simulink model "AvonGasTurbineDgTwin"  (R2024b)
settings: Solver=VariableStepAuto  StartTime=0  StopTime=7200  FixedStep=1  RelTol=1e-3  EnableMultiTasking=on
InitFcn:
  | warning off
undefined symbols (not defined in the file or in its folder): ENV_ambient_moisture_pct, ENV_comp_inlet_press_kPa, ENV_comp_inlet_temp_C, ENV_FG_pressure_kPa, ENV_FG_temp_C
libraries: slpidlib x3, simulink x2
(part 3 of 3)

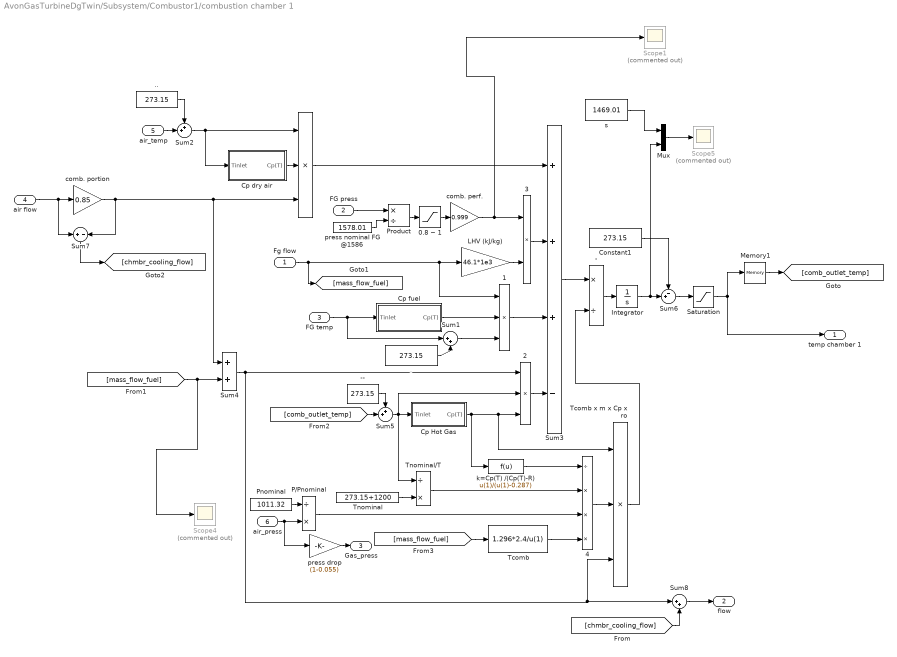
== system AvonGasTurbineDgTwin/Subsystem/Combustor1/combustion chamber 1 ==
  Fg flow : Inport
  FG press : Inport  Port=2
  FG temp : Inport  Port=3
  air flow : Inport  Port=4
  air_temp : Inport  Port=5
  air_press : Inport  Port=6
  "     " : Product  Inputs=3  RndMeth=Zero
  "     1" : Product  Inputs=3  RndMeth=Zero
  "     2" : Product  Inputs=3  RndMeth=Zero
  "     3" : Product  RndMeth=Zero
  "     4" : Product  Inputs=/***  RndMeth=Zero
  " Cp dry air " : Subsystem
  - : Product  Inputs=*/  RndMeth=Zero
  -- : Constant  Value=273.15
  . : Constant  Value=273.15
  .. : Constant  Value=273.15
  0.8 ~ 1 : Saturate  UpperLimit=1  LowerLimit=0.8
  Constant1 : Constant  Value=273.15
  "Cp Hot Gas " : Subsystem
  Cp fuel : Subsystem
  Integrator : Integrator  InitialCondition=780+273.15  LimitOutput=on  UpperSaturationLimit=2000  LowerSaturationLimit=780+273.15
  "LHV (kJ/kg) " : Gain  Gain=46.1*1e3
  Memory1 : Memory  InitialCondition=780
  Mux : Mux  Inputs=2
  P/Pnominal : Product  Inputs=/*  RndMeth=Zero
  Pnominal : Constant  Value=1011.32
  Product : Product  Inputs=*/
  Saturation : Saturate  UpperLimit=1400  LowerLimit=350
  Scope1 : Scope  Commented=on
  Scope4 : Scope  Commented=on
  Scope5 : Scope  Commented=on
  Sum1 : Sum  Inputs=|++
  Sum2 : Sum  Inputs=++|
  Sum3 : Sum  Inputs=+++-
  Sum4 : Sum  Inputs=2
  Sum5 : Sum  Inputs=++|
  Sum6 : Sum  Inputs=-+|
  Sum7 : Sum  Inputs=+-
  Sum8 : Sum  Inputs=|++
  Tcomb : Fcn  Expr=1.296*2.4/u(1)  SampleTime=1
  Tcomb x m x Cp x ro : Product  Inputs=3  RndMeth=Zero
  Tnominal : Constant  Value=273.15+1200
  Tnominal/T : Product  Inputs=/*  RndMeth=Zero
  comb. perf. : Gain  Gain=0.999
  comb. portion : Gain  Gain=0.85
  k=Cp(T) /(Cp(T)-R) : Fcn  Expr=u(1)/(u(1)-0.287)
  press drop : Gain  Gain=(1-0.055)  SampleTime=1
  press nominal FG @1586 : Constant  Value=1578.01
  s : Constant  Value=1469.01
  temp chamber 1 : Outport
  flow : Outport  Port=2
  Gas_press : Outport  Port=3
  wires:
  " Cp dry air "/1(Cp(T)) -> "     "/2
  ../1 -> Sum2/1
  Sum2/1 -> " Cp dry air "/1(Tinlet), "     "/1
  FG press/1 -> Product/1
  FG temp/1 -> Sum1/1, Cp fuel/1(Tinlet)
  Sum3/1 -> -/1
  Fg flow/1 -> "     1"/1, "LHV (kJ/kg) "/1, [mass_flow_fuel]
  Sum1/1 -> "     1"/3
  Cp fuel/1(Cp(T)) -> "     1"/2
  "     "/1 -> Sum3/1
  Memory1/1 -> [comb_outlet_temp]
  "     1"/1 -> Sum3/3
  ./1 -> Sum1/2
  "     2"/1 -> Sum3/4
  Tnominal/1 -> Tnominal/T/2
  Sum5/1 -> "     2"/2, "Cp Hot Gas "/1(Tinlet), Tnominal/T/1
  Constant1/1 -> Sum6/1
  Integrator/1 -> Mux/2, Sum6/2
  Sum6/1 -> Saturation/1
  "LHV (kJ/kg) "/1 -> "     3"/2
  Tcomb x m x Cp x ro/1 -> -/2
  Tnominal/T/1 -> "     4"/2
  [mass_flow_fuel] -> Scope4/1, Sum4/2
  "Cp Hot Gas "/1(Cp(T)) -> k=Cp(T) /(Cp(T)-R)/1, "     2"/3, Tcomb x m x Cp x ro/1
  --/1 -> Sum5/1
  Pnominal/1 -> P/Pnominal/1
  air_press/1 -> press drop/1, P/Pnominal/2
  "     4"/1 -> Tcomb x m x Cp x ro/2
  k=Cp(T) /(Cp(T)-R)/1 -> "     4"/1
  [comb_outlet_temp] -> Sum5/2
  P/Pnominal/1 -> "     4"/3
  air_temp/1 -> Sum2/2
  -/1 -> Integrator/1
  Saturation/1 -> temp chamber 1/1, Memory1/1
  s/1 -> Mux/1
  Sum4/1 -> "     2"/1, Sum8/1, Tcomb x m x Cp x ro/3
  Mux/1 -> Scope5/1
  press drop/1 -> Gas_press/1
  press nominal FG @1586/1 -> Product/2
  Product/1 -> 0.8 ~ 1/1
  0.8 ~ 1/1 -> comb. perf./1
  comb. perf./1 -> "     3"/1, Scope1/1
  "     3"/1 -> Sum3/2
  [mass_flow_fuel] -> Tcomb/1
  Tcomb/1 -> "     4"/4
  air flow/1 -> Sum7/1, comb. portion/1
  comb. portion/1 -> Sum7/2, "     "/3, Sum4/1
  Sum8/1 -> flow/1
  [chmbr_cooling_flow] -> Sum8/2
  Sum7/1 -> [chmbr_cooling_flow]

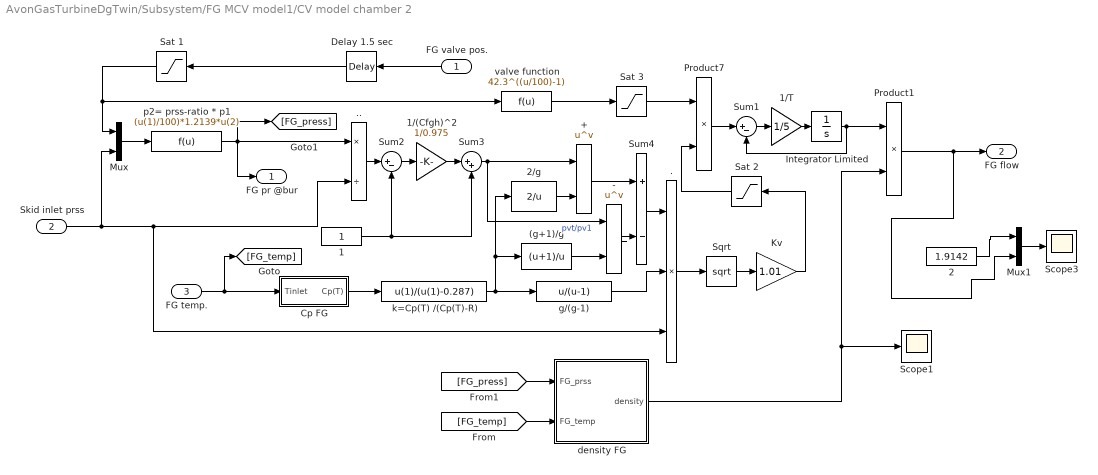
== system AvonGasTurbineDgTwin/Subsystem/FG MCV model1/CV model chamber 2 ==
  FG valve pos. : Inport
  Skid inlet prss : Inport  Port=2
  FG temp. : Inport  Port=3
  "  (g+1)/g" : Fcn  Expr=(u+1)/u
  "  Sqrt  " : Sqrt
  " k=Cp(T) /(Cp(T)-R) " : Fcn  Expr=u(1)/(u(1)-0.287)
  + : Math  Operator=pow  SignedPower=on
  - : Math  Operator=pow  SignedPower=on
  . : Product  Inputs=3  RndMeth=Zero
  .. : Product  Inputs=*/  RndMeth=Zero
  1 : Constant
  1/(Cfgh)^2 : Gain  Gain=1/0.975
  1/T : Gain  Gain=1/5
  2 : Constant  Value=1.9142
  2/g : Fcn  Expr=2/u
  Cp FG : Subsystem
  Delay 1.5 sec : TransportDelay  DelayTime=1.5  InitialOutput=30
  Integrator Limited : Integrator  InitialCondition=1.9  LimitOutput=on  UpperSaturationLimit=5  LowerSaturationLimit=0.01
  Kv : Gain  Gain=1.01
  Mux : Mux  Inputs=2
  Mux1 : Mux  Inputs=2
  Product1 : Product  RndMeth=Zero
  Product7 : Product  RndMeth=Zero
  Sat 1 : Saturate  UpperLimit=100  LowerLimit=0.01
  Sat 2 : Saturate  UpperLimit=300  LowerLimit=0.001
  Sat 3 : Saturate  UpperLimit=1  LowerLimit=0.01
  Scope1 : Scope
  Scope3 : Scope
  Sum1 : Sum  Inputs=|+-
  Sum2 : Sum  Inputs=|+-
  Sum3 : Sum  Inputs=|++
  Sum4 : Sum  Inputs=+-
  density FG : Subsystem
  g/(g-1) : Fcn  Expr=u/(u-1)
  p2= prss-ratio * p1 : Fcn  Expr=(u(1)/100)*1.2139*u(2)  SampleTime=1
  valve function : Fcn  Expr=42.3^((u/100)-1)  SampleTime=1
  FG pr @bur : Outport
  FG flow : Outport  Port=2
  wires:
  Sat 2/1 -> Product7/2
  Sum3/1 -> +/1, -/1  "pvt/pv1"
  Sum4/1 -> ./1
  "  Sqrt  "/1 -> Kv/1
  ../1 -> Sum2/1
  Skid inlet prss/1 -> ../2, ./3, Mux/2
  2/g/1 -> +/2
  1/(Cfgh)^2/1 -> Sum3/1
  Sum2/1 -> 1/(Cfgh)^2/1
  FG temp./1 -> [FG_temp], Cp FG/1(Tinlet)
  "  (g+1)/g"/1 -> -/2
  -/1 -> Sum4/2
  " k=Cp(T) /(Cp(T)-R) "/1 -> g/(g-1)/1, "  (g+1)/g"/1, 2/g/1
  g/(g-1)/1 -> ./2
  p2= prss-ratio * p1/1 -> [FG_press], ../1, FG pr @bur/1
  +/1 -> Sum4/1
  1/1 -> Sum3/2, Sum2/2
  Cp FG/1(Cp(T)) -> " k=Cp(T) /(Cp(T)-R) "/1
  Mux/1 -> p2= prss-ratio * p1/1
  valve function/1 -> Sat 3/1
  FG valve pos./1 -> Delay 1.5 sec/1
  Delay 1.5 sec/1 -> Sat 1/1
  Sat 1/1 -> Mux/1, valve function/1
  Sat 3/1 -> Product7/1
  Kv/1 -> Sat 2/1
  Sum1/1 -> 1/T/1
  1/T/1 -> Integrator Limited/1
  Integrator Limited/1 -> Product1/1, Sum1/2
  ./1 -> "  Sqrt  "/1
  Product7/1 -> Sum1/1
  [FG_temp] -> density FG/2(FG_temp)
  [FG_press] -> density FG/1(FG_prss)
  density FG/1(density) -> Scope1/1, Product1/2
  Mux1/1 -> Scope3/1
  Product1/1 -> Mux1/2, FG flow/1
  2/1 -> Mux1/1

== system AvonGasTurbineDgTwin/Subsystem/FG MCV model1/FAULT_07_FuelPrssRegulatorStuck ==
  main FG line prss : Inport
  FAULT_07_multiplier : FromWorkspace  VariableName=FAULT_07_multiplier  SampleTime=-1
  Mux : Mux  Inputs=2
  Product : Product
  Scope{,1..3} (4 alike) : Scope  Commented=on
  Out1 : Outport
  wires:
  FAULT_07_multiplier/1 -> Product/1, Scope/1
  main FG line prss/1 -> Scope1/1, Mux/2, Product/2
  Product/1 -> Mux/1, Scope2/1, Out1/1
  Mux/1 -> Scope3/1

== system AvonGasTurbineDgTwin/Subsystem/FG MCV model1/FAULT_08_FuelValveLeakage ==
  In1 : Inport
  FAULT_08_multiplier : FromWorkspace  VariableName=FAULT_08_multiplier  SampleTime=-1
  Mux : Mux  Inputs=2
  Product : Product
  Scope{,1..3} (4 alike) : Scope  Commented=on
  Out1 : Outport
  wires:
  FAULT_08_multiplier/1 -> Product/1, Scope/1
  In1/1 -> Scope1/1, Mux/2, Product/2
  Product/1 -> Mux/1, Scope2/1, Out1/1
  Mux/1 -> Scope3/1

== system AvonGasTurbineDgTwin/Subsystem/FG MCV model1/FAULT_09_FuelContamination ==
  In1 : Inport
  FAULT_09_multiplier : FromWorkspace  VariableName=FAULT_09_multiplier  SampleTime=-1
  Mux : Mux  Inputs=2
  Product : Product
  Scope{,1..3} (4 alike) : Scope  Commented=on
  Out1 : Outport
  wires:
  FAULT_09_multiplier/1 -> Product/1, Scope/1
  In1/1 -> Scope1/1, Mux/2, Product/2
  Product/1 -> Mux/1, Scope2/1, Out1/1
  Mux/1 -> Scope3/1

== system AvonGasTurbineDgTwin/Subsystem/FG MCV model1/FAULT_10_FuelLineBlockage ==
  In1 : Inport
  FAULT_10_multiplier : FromWorkspace  VariableName=FAULT_10_multiplier  SampleTime=-1
  Mux : Mux  Inputs=2
  Product : Product
  Scope{,1..3} (4 alike) : Scope  Commented=on
  Out1 : Outport
  wires:
  FAULT_10_multiplier/1 -> Product/1, Scope/1
  In1/1 -> Scope1/1, Mux/2, Product/2
  Product/1 -> Mux/1, Scope2/1, Out1/1
  Mux/1 -> Scope3/1

== system AvonGasTurbineDgTwin/Subsystem/FG MCV model1/FAULT_11_FuelPumpDegradation ==
  In1 : Inport
  FAULT_11_multiplier : FromWorkspace  VariableName=FAULT_11_multiplier  SampleTime=-1
  Mux : Mux  Inputs=2
  Product : Product
  Scope{,1..3} (4 alike) : Scope  Commented=on
  Out1 : Outport
  wires:
  FAULT_11_multiplier/1 -> Product/1, Scope/1
  In1/1 -> Scope1/1, Mux/2, Product/2
  Product/1 -> Mux/1, Scope2/1, Out1/1
  Mux/1 -> Scope3/1

== system AvonGasTurbineDgTwin/Subsystem/FG MCV model1/FAULT_12_FuelSupplyPressDrop ==
  In1 : Inport
  FAULT_12_multiplier : FromWorkspace  VariableName=FAULT_12_multiplier  SampleTime=-1
  Mux : Mux  Inputs=2
  Product : Product
  Scope{,1..3} (4 alike) : Scope  Commented=on
  Out1 : Outport
  wires:
  FAULT_12_multiplier/1 -> Product/1, Scope/1
  In1/1 -> Scope1/1, Mux/2, Product/2
  Product/1 -> Mux/1, Scope2/1, Out1/1
  Mux/1 -> Scope3/1

== system AvonGasTurbineDgTwin/Subsystem/FG MCV model1/FAULT_13_FGSupplyPressOscillation ==
  In1 : Inport
  FAULT_13_multiplier : FromWorkspace  VariableName=FAULT_13_multiplier  SampleTime=-1
  Mux : Mux  Inputs=2
  Product : Product
  Scope{,1..3} (4 alike) : Scope  Commented=on
  Out1 : Outport
  wires:
  FAULT_13_multiplier/1 -> Product/1, Scope/1
  In1/1 -> Scope1/1, Mux/2, Product/2
  Product/1 -> Mux/1, Scope2/1, Out1/1
  Mux/1 -> Scope3/1

== system AvonGasTurbineDgTwin/Subsystem/FG MCV model1/FAULT_16_FuelValveLeak ==
  FG flow : Inport
  FAULT_16_multiplier : FromWorkspace  VariableName=FAULT_16_multiplier  SampleTime=-1
  Mux : Mux  Inputs=2
  Product : Product
  Scope{,1..3} (4 alike) : Scope  Commented=on
  Out1 : Outport
  wires:
  FAULT_16_multiplier/1 -> Product/1, Scope/1
  FG flow/1 -> Scope1/1, Mux/2, Product/2
  Product/1 -> Mux/1, Scope2/1, Out1/1
  Mux/1 -> Scope3/1

== system AvonGasTurbineDgTwin/Subsystem/FG MCV model1/Subsystem1 ==
  gas prss : Inport
  FG temp. : Inport  Port=2
  FG flow : Inport  Port=3
  " 2 " : Constant  Value=2
  . : Product  Inputs=3  RndMeth=Zero
  2 : Constant  Value=2
  Kf : Gain  Gain=16.8993
  Math Function5 : Math  Operator=pow  SignedPower=on
  Memory : Memory
  Sqrt : Sqrt
  Sqrt1 : Sqrt
  Sqrt2 : Sqrt
  Sum1 : Sum  Inputs=-+|
  Sum5 : Sum  Inputs=|++
  Sum9 : Sum  Inputs=|+-
  Z : Subsystem
  c4 : Constant  Value=273.15
  n flow exp. : Constant  Value=0.4835
  pressure drop 5 kPa : Constant  Value=5
  pw : Math  Operator=pow  SignedPower=on
  pw1 : Math  Operator=pow  SignedPower=on
  " FG skid inlet prss" : Outport
  skid temp : Outport  Port=2
  wires:
  pressure drop 5 kPa/1 -> Sum1/1
  Sum1/1 -> pw1/1
  Sqrt1/1 -> ./3
  Memory/1 -> Z/2(P)
  Sqrt/1 -> ./2
  Sum5/1 -> Z/1(T), Sqrt/1
  c4/1 -> Sum5/2
  Z/1(Z) -> Sqrt1/1
  Sqrt2/1 -> Memory/1, " FG skid inlet prss"/1
  Math Function5/1 -> ./1
  FG flow/1 -> Math Function5/1
  n flow exp./1 -> Math Function5/2
  pw/1 -> Sum9/2
  2/1 -> pw/2
  Sum9/1 -> Sqrt2/1
  pw1/1 -> Sum9/1
  Kf/1 -> pw/1
  ./1 -> Kf/1
  FG temp./1 -> Sum5/1, skid temp/1
  " 2 "/1 -> pw1/2
  gas prss/1 -> Sum1/2

== system AvonGasTurbineDgTwin/Subsystem/GasGenerator/Cp @ trb. input ==
  Tinlet : Inport
  Cp : Fcn  Expr=(3.355+5.75*1e-4*u(1)-1600*u(1)^(-2))*0.28714  SampleTime=1
  Cp(T) : Outport
  wires:
  Tinlet/1 -> Cp/1
  Cp/1 -> Cp(T)/1

== system AvonGasTurbineDgTwin/Subsystem/GasGenerator/Cp @ trb. output ==
  Tinlet : Inport
  Cp : Fcn  Expr=(3.355+5.75*1e-4*u(1)-1600*u(1)^(-2))*0.28714  SampleTime=1
  Cp(T) : Outport
  wires:
  Cp/1 -> Cp(T)/1
  Tinlet/1 -> Cp/1

== system AvonGasTurbineDgTwin/Subsystem/GasGenerator/FAULT_23_GGNozzleBlockage ==
  hot_gas_flow : Inport
  FAULT_23_multiplier : FromWorkspace  VariableName=FAULT_23_multiplier  SampleTime=-1
  Mux : Mux  Inputs=2
  Product : Product
  Scope{,1..3} (4 alike) : Scope  Commented=on
  Out1 : Outport
  wires:
  FAULT_23_multiplier/1 -> Product/1, Scope/1
  hot_gas_flow/1 -> Scope1/1, Mux/2, Product/2
  Product/1 -> Mux/1, Scope2/1, Out1/1
  Mux/1 -> Scope3/1

== system AvonGasTurbineDgTwin/Subsystem/GasGenerator/FAULT_24_GGSealDegradation ==
  rotor_cooling_air_flow : Inport
  FAULT_24_multiplier : FromWorkspace  VariableName=FAULT_24_multiplier  SampleTime=-1
  Mux : Mux  Inputs=2
  Product : Product
  Scope{,1..3} (4 alike) : Scope  Commented=on
  Out1 : Outport
  wires:
  FAULT_24_multiplier/1 -> Product/1, Scope/1
  rotor_cooling_air_flow/1 -> Scope1/1, Mux/2, Product/2
  Product/1 -> Mux/1, Scope2/1, Out1/1
  Mux/1 -> Scope3/1

== system AvonGasTurbineDgTwin/Subsystem/GasGenerator/FAULT_33_SensorEnhancement ==
  In1 : Inport
  FAULT_33_multiplier : FromWorkspace  VariableName=FAULT_33_multiplier  SampleTime=-1
  Mux : Mux  Inputs=2
  Product : Product
  Scope{,1..3} (4 alike) : Scope  Commented=on
  Out1 : Outport
  wires:
  FAULT_33_multiplier/1 -> Product/1, Scope/1
  In1/1 -> Scope1/1, Mux/2, Product/2
  Product/1 -> Mux/1, Scope2/1, Out1/1
  Mux/1 -> Scope3/1

== system AvonGasTurbineDgTwin/Subsystem/GasGenerator/FAULT_34_SensorDegradation ==
  In1 : Inport
  FAULT_34_multiplier : FromWorkspace  VariableName=FAULT_34_multiplier  SampleTime=-1
  Mux : Mux  Inputs=2
  Product : Product
  Scope{,1..3} (4 alike) : Scope  Commented=on
  Out1 : Outport
  wires:
  FAULT_34_multiplier/1 -> Product/1, Scope/1
  In1/1 -> Scope1/1, Mux/2, Product/2
  Product/1 -> Mux/1, Scope2/1, Out1/1
  Mux/1 -> Scope3/1

== system AvonGasTurbineDgTwin/Subsystem/GasGenerator/FAULT_35_SensorEnhanceStep ==
  In1 : Inport
  FAULT_35_multiplier : FromWorkspace  VariableName=FAULT_35_multiplier  SampleTime=-1
  Mux : Mux  Inputs=2
  Product : Product
  Scope{,1..3} (4 alike) : Scope  Commented=on
  Out1 : Outport
  wires:
  FAULT_35_multiplier/1 -> Product/1, Scope/1
  In1/1 -> Scope1/1, Mux/2, Product/2
  Product/1 -> Mux/1, Scope2/1, Out1/1
  Mux/1 -> Scope3/1

== system AvonGasTurbineDgTwin/Subsystem/GasGenerator/FAULT_36_SensorDegradeStep ==
  In1 : Inport
  FAULT_36_multiplier : FromWorkspace  VariableName=FAULT_36_multiplier  SampleTime=-1
  Mux : Mux  Inputs=2
  Product : Product
  Scope{,1..3} (4 alike) : Scope  Commented=on
  Out1 : Outport
  wires:
  FAULT_36_multiplier/1 -> Product/1, Scope/1
  In1/1 -> Scope1/1, Mux/2, Product/2
  Product/1 -> Mux/1, Scope2/1, Out1/1
  Mux/1 -> Scope3/1

== system AvonGasTurbineDgTwin/Subsystem/GasGenerator/FAULT_37_SensorFreez ==
  temp gas : Inport
  FAULT_37_multiplier : FromWorkspace  VariableName=FAULT_37_multiplier  SampleTime=-1
  Memory : Memory  InheritSampleTime=on
  Scope{,1..3} (4 alike) : Scope  Commented=on
  Switch : Switch  Criteria=u2 > Threshold  Threshold=0.5  SaturateOnIntegerOverflow=off  InputSameDT=off
  Out1 : Outport
  wires:
  FAULT_37_multiplier/1 -> Scope3/1, Switch/2
  temp gas/1 -> Scope2/1, Switch/1
  Memory/1 -> Scope/1, Switch/3
  Switch/1 -> Scope1/1, Out1/1, Memory/1

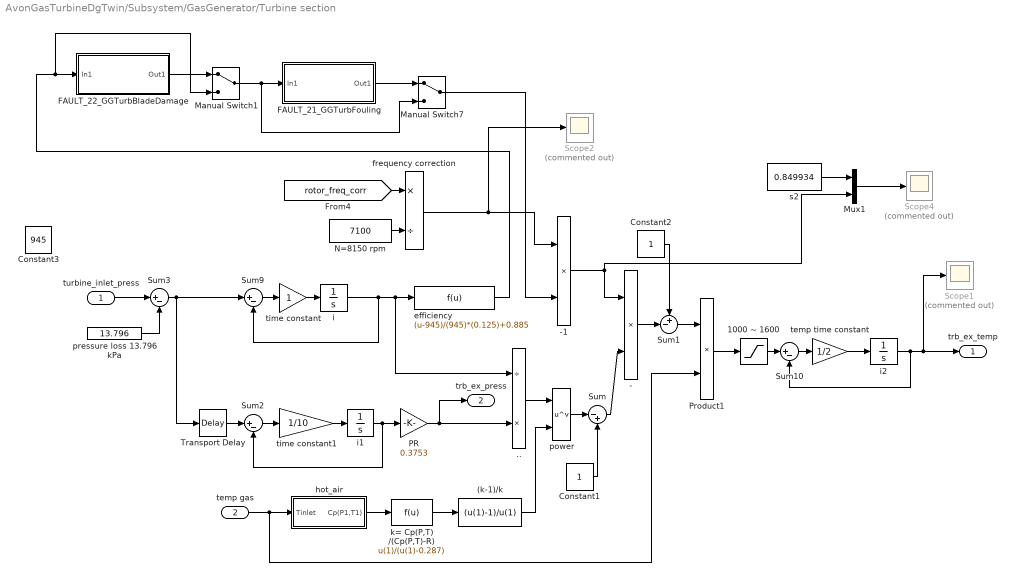
== system AvonGasTurbineDgTwin/Subsystem/GasGenerator/Turbine section ==
  turbine_inlet_press : Inport
  temp gas : Inport  Port=2
  (k-1)/k : Fcn  Expr=(u(1)-1)/u(1)
  - : Product  RndMeth=Zero
  -1 : Product  RndMeth=Zero
  .. : Product  Inputs=/*  RndMeth=Zero
  1000 ~ 1600 : Saturate  UpperLimit=2000  LowerLimit=400
  Constant1 : Constant
  Constant2 : Constant
  Constant3 : Constant  Value=945
  FAULT_21_GGTurbFouling : Subsystem
  FAULT_22_GGTurbBladeDamage : Subsystem
  Manual Switch1 : ManualSwitch
  Manual Switch7 : ManualSwitch
  Mux1 : Mux  Inputs=2
  N=8150 rpm : Constant  Value=7100
  PR : Gain  Gain=0.3753
  Product1 : Product  RndMeth=Zero
  Scope1 : Scope  Commented=on
  Scope2 : Scope  Commented=on
  Scope4 : Scope  Commented=on
  Sum : Sum  Inputs=|-+
  Sum1 : Sum  Inputs=+-|
  Sum{2..3,9..10} (4 alike) : Sum  Inputs=|+-
  Transport Delay : TransportDelay  DelayTime=1.6  InitialOutput=941.9108
  efficiency : Fcn  Expr=(u-945)/(945)*(0.125)+0.885
  frequency correction : Product  Inputs=*/  RndMeth=Zero
  hot_air : Subsystem
  i : Integrator  InitialCondition=507  LimitOutput=on  UpperSaturationLimit=1100  LowerSaturationLimit=10
  i1 : Integrator  InitialCondition=507  LimitOutput=on  UpperSaturationLimit=1100  LowerSaturationLimit=500
  i2 : Integrator  InitialCondition=450+273.15  LimitOutput=on  UpperSaturationLimit=2000  LowerSaturationLimit=400
  k= Cp(P,T) /(Cp(P,T)-R) : Fcn  Expr=u(1)/(u(1)-0.287)
  power : Math  Operator=pow  SignedPower=on
  pressure loss 13.796 kPa : Constant  Value=13.796
  s2 : Constant  Value=0.849934
  temp time constant : Gain  Gain=1/2
  time constant : Gain
  time constant1 : Gain  Gain=1/10
  trb_ex_temp : Outport
  trb_ex_press : Outport  Port=2
  wires:
  i/1 -> Sum9/2, efficiency/1, ../1
  power/1 -> Sum/1
  Constant1/1 -> Sum/2
  -/1 -> Sum1/2
  Sum3/1 -> Sum9/1, Transport Delay/1
  k= Cp(P,T) /(Cp(P,T)-R)/1 -> (k-1)/k/1
  hot_air/1(Cp(P1,T1)) -> k= Cp(P,T) /(Cp(P,T)-R)/1
  (k-1)/k/1 -> power/2
  Sum/1 -> -/2
  Sum9/1 -> time constant/1
  time constant/1 -> i/1
  Sum10/1 -> temp time constant/1
  temp time constant/1 -> i2/1
  Product1/1 -> 1000 ~ 1600/1
  pressure loss 13.796 kPa/1 -> Sum3/2
  Constant2/1 -> Sum1/1
  Sum1/1 -> Product1/1
  temp gas/1 -> hot_air/1(Tinlet), Product1/2
  1000 ~ 1600/1 -> Sum10/1
  i2/1 -> Scope1/1, trb_ex_temp/1, Sum10/2
  Mux1/1 -> Scope4/1
  s2/1 -> Mux1/1
  -1/1 -> -/1, Mux1/2
  i1/1 -> Sum2/2, PR/1
  Sum2/1 -> time constant1/1
  time constant1/1 -> i1/1
  turbine_inlet_press/1 -> Sum3/1
  PR/1 -> trb_ex_press/1, ../2
  ../1 -> power/1
  Transport Delay/1 -> Sum2/1
  N=8150 rpm/1 -> frequency correction/2
  [rotor_freq_corr] -> frequency correction/1
  frequency correction/1 -> Scope2/1, -1/1
  FAULT_21_GGTurbFouling/1(Out1) -> Manual Switch7/1
  Manual Switch7/1 -> -1/2
  FAULT_22_GGTurbBladeDamage/1(Out1) -> Manual Switch1/1
  efficiency/1 -> Manual Switch1/2, FAULT_22_GGTurbBladeDamage/1(In1)
  Manual Switch1/1 -> Manual Switch7/2, FAULT_21_GGTurbFouling/1(In1)

== system AvonGasTurbineDgTwin/Subsystem/GasGenerator/cooling 1 ==
  cooling_air_temp : Inport
  cooling_air_flow : Inport  Port=2
  hot_gas_flow : Inport  Port=3
  hot_gas_temp : Inport  Port=4
  "     1" : Product  RndMeth=Zero
  "     2" : Product  Inputs=3  RndMeth=Zero
  "     4" : Product  Inputs=3  RndMeth=Zero
  . : Product  Inputs=*/  RndMeth=Zero
  Cp Temp : Subsystem
  Cp Temp air : Subsystem
  Cp Temp hot gas : Subsystem
  Integrator : Integrator  InitialCondition=765+273.15+12  LimitOutput=on  UpperSaturationLimit=1250+273.15  LowerSaturationLimit=600+273.15
  Memory : Memory  InitialCondition=750+273.15
  Scope1 : Scope  Commented=on
  Sum1 : Sum  Inputs=2
  Sum2 : Sum  Inputs=2
  Sum6 : Sum  Inputs=|+-
  time constant : Gain  Gain=1/3.6
  temp gas : Outport
  gas_flow : Outport  Port=2
  wires:
  hot_gas_temp/1 -> Cp Temp hot gas/1(Tinlet), "     4"/2
  hot_gas_flow/1 -> Sum1/1, "     4"/1
  Cp Temp hot gas/1(Cp(T)) -> "     4"/3
  cooling_air_temp/1 -> Cp Temp air/1(Tinlet), "     2"/2
  cooling_air_flow/1 -> Sum1/2, "     2"/1
  Cp Temp air/1(Cp(T)) -> "     2"/3
  "     2"/1 -> Sum2/1
  "     4"/1 -> Sum2/2
  Sum2/1 -> ./1
  Cp Temp/1(Cp(T)) -> "     1"/2
  Memory/1 -> Cp Temp/1(Tinlet)
  "     1"/1 -> ./2
  ./1 -> Sum6/1
  time constant/1 -> Integrator/1
  Sum6/1 -> time constant/1
  Integrator/1 -> temp gas/1, Scope1/1, Sum6/2, Memory/1
  Sum1/1 -> "     1"/1, gas_flow/1

== system AvonGasTurbineDgTwin/Subsystem/GasGenerator/cooling 2 ==
  cooling_air_temp : Inport
  cooling_air_flow : Inport  Port=2
  hot_gas_flow : Inport  Port=3
  hot_gas_temp : Inport  Port=4
  "     1" : Product  RndMeth=Zero
  "     2" : Product  Inputs=3  RndMeth=Zero
  "     4" : Product  Inputs=3  RndMeth=Zero
  . : Product  Inputs=*/  RndMeth=Zero
  Constant : Constant  Value=-600
  Cp Temp : Subsystem
  Cp Temp air : Subsystem
  Cp Temp hot gas : Subsystem
  Integrator : Integrator  InitialCondition=1204.4  LimitOutput=on  UpperSaturationLimit=2000  LowerSaturationLimit=100
  Memory : Memory  InitialCondition=500+273.15
  Scope1 : Scope  Commented=on
  Scope4 : Scope  Commented=on
  Sum1 : Sum  Inputs=2
  Sum2 : Sum  Inputs=2
  Sum3 : Sum  Inputs=++|
  Sum6 : Sum  Inputs=|+-
  Sum7 : Sum  Inputs=|++
  offset compensator1 : Fcn  Expr=(u-87)/(87)*(14.48)-14.45
  time constant : Gain  Gain=1/5
  gas_flow : Outport
  temp turb : Outport  Port=2
  temp exh turb : Outport  Port=3
  wires:
  Sum6/1 -> time constant/1
  time constant/1 -> Integrator/1
  ./1 -> Sum6/1
  "     1"/1 -> ./2
  Memory/1 -> Cp Temp/1(Tinlet)
  Cp Temp/1(Cp(T)) -> "     1"/2
  Sum1/1 -> Scope4/1, gas_flow/1, "     1"/1, offset compensator1/1
  Sum2/1 -> ./1
  "     4"/1 -> Sum2/2
  "     2"/1 -> Sum2/1
  Cp Temp air/1(Cp(T)) -> "     2"/3
  cooling_air_flow/1 -> "     2"/1, Sum1/2
  cooling_air_temp/1 -> "     2"/2, Cp Temp air/1(Tinlet)
  Cp Temp hot gas/1(Cp(T)) -> "     4"/3
  hot_gas_flow/1 -> "     4"/1, Sum1/1
  hot_gas_temp/1 -> "     4"/2, Cp Temp hot gas/1(Tinlet), Sum3/1
  Integrator/1 -> Sum7/1, Scope1/1, Sum6/2, Memory/1
  Sum3/1 -> temp turb/1
  offset compensator1/1 -> Sum3/2
  Sum7/1 -> temp exh turb/1

== system AvonGasTurbineDgTwin/Subsystem/GasGenerator/rotor dynamic  ==
  gen_turb : Inport
  consm_comp : Inport  Port=2
  ...1 : Product  Inputs=*/
  ...2 : Product  Inputs=/*
  ...3 : Product
  F1 : Constant  Value=1.9141
  Gain1 : Gain  Gain=0.5
  Gain2 : Gain  Gain=30/pi
  Gain4 : Gain  Gain=pi/30
  Integrator1 : Integrator  InitialCondition=pi/30*7250  LimitOutput=on  UpperSaturationLimit=1200  LowerSaturationLimit=0.01
  J_rotor1 : Gain  Gain=1/60
  Loss : Gain  Gain=0.001
  Math Function : Math  Operator=square  SignedPower=on
  Memory Omega2 : Memory  InitialCondition=pi/30*7250
  Mux4 : Mux  Inputs=2
  Product2 : Product  Inputs=*/
  Scope1 : Scope  Commented=on
  Scope8 : Scope  Commented=on
  Scope9 : Scope  Commented=on
  Sum1 : Sum  Inputs=++|
  Sum7 : Sum  Inputs=|++
  Sum8 : Sum  Inputs=|+-
  Sum9 : Sum  Inputs=|+-
  freq_rotor2 : Constant
  freq_rotor3 : Constant  Value=7250
  power1 : Constant  Value=7250
  rotor_speed : Outport
  wires:
  F1/1 -> Product2/2
  Memory Omega2/1 -> Sum7/2
  Gain4/1 -> ...2/1, Sum7/1
  Sum7/1 -> ...2/2, ...1/2
  [FG_flow] -> Product2/1
  freq_rotor3/1 -> Gain4/1
  J_rotor1/1 -> Integrator1/1
  Loss/1 -> Sum9/2
  consm_comp/1 -> Sum8/2
  ...2/1 -> Math Function/1
  Math Function/1 -> Loss/1
  power1/1 -> Mux4/2
  Mux4/1 -> Scope9/1
  Gain2/1 -> Mux4/1
  gen_turb/1 -> Sum8/1
  Sum9/1 -> ...1/1
  ...1/1 -> ...3/2
  Product2/1 -> Sum1/1
  Gain1/1 -> Scope1/1, ...3/1
  freq_rotor2/1 -> Sum1/2
  Sum1/1 -> Gain1/1
  ...3/1 -> J_rotor1/1
  Integrator1/1 -> Memory Omega2/1, Gain2/1, rotor_speed/1
  Sum8/1 -> Scope8/1, Sum9/1

== system AvonGasTurbineDgTwin/Subsystem/PowerTurbine/Cp @ trb. input ==
  Tinlet : Inport
  Cp : Fcn  Expr=(3.355+5.75*1e-4*u(1)-1600*u(1)^(-2))*0.28714  SampleTime=1
  Cp(T) : Outport
  wires:
  Cp/1 -> Cp(T)/1
  Tinlet/1 -> Cp/1

== system AvonGasTurbineDgTwin/Subsystem/PowerTurbine/Cp @ trb. output ==
  Tinlet : Inport
  Cp : Fcn  Expr=(3.355+5.75*1e-4*u(1)-1600*u(1)^(-2))*0.28714  SampleTime=1
  Cp(T) : Outport
  wires:
  Tinlet/1 -> Cp/1
  Cp/1 -> Cp(T)/1

== system AvonGasTurbineDgTwin/Subsystem/PowerTurbine/FAULT_28_PTNozzleDamage ==
  hot_gas_flow : Inport
  FAULT_28_multiplier : FromWorkspace  VariableName=FAULT_28_multiplier  SampleTime=-1
  Mux : Mux  Inputs=2
  Product : Product
  Scope{,1..3} (4 alike) : Scope  Commented=on
  Out1 : Outport
  wires:
  FAULT_28_multiplier/1 -> Product/1, Scope/1
  hot_gas_flow/1 -> Scope1/1, Mux/2, Product/2
  Product/1 -> Mux/1, Scope2/1, Out1/1
  Mux/1 -> Scope3/1

== system AvonGasTurbineDgTwin/Subsystem/PowerTurbine/FAULT_31_PTPowerLoss ==
  In1 : Inport
  FAULT_31_multiplier : FromWorkspace  VariableName=FAULT_31_multiplier  SampleTime=-1
  Mux : Mux  Inputs=2
  Product : Product
  Scope{,1..3} (4 alike) : Scope  Commented=on
  Out1 : Outport
  wires:
  FAULT_31_multiplier/1 -> Product/1, Scope/1
  In1/1 -> Scope1/1, Mux/2, Product/2
  Product/1 -> Mux/1, Scope2/1, Out1/1
  Mux/1 -> Scope3/1

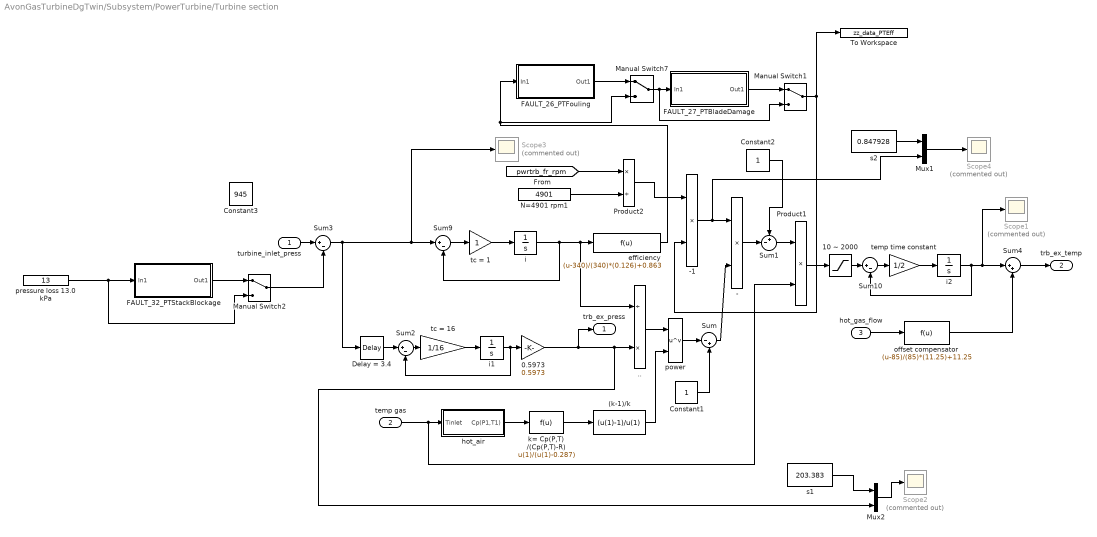
== system AvonGasTurbineDgTwin/Subsystem/PowerTurbine/Turbine section ==
  turbine_inlet_press : Inport
  temp gas : Inport  Port=2
  hot_gas_flow : Inport  Port=3
  (k-1)/k : Fcn  Expr=(u(1)-1)/u(1)
  - : Product  RndMeth=Zero
  -1 : Product  RndMeth=Zero
  .. : Product  Inputs=/*  RndMeth=Zero
  0.5973 : Gain  Gain=0.5973
  10 ~ 2000 : Saturate  UpperLimit=2000  LowerLimit=10
  Constant1 : Constant
  Constant2 : Constant
  Constant3 : Constant  Value=945
  Delay = 3.4 : TransportDelay  DelayTime=3.4  InitialOutput=230.380
  FAULT_26_PTFouling : Subsystem
  FAULT_27_PTBladeDamage : Subsystem
  FAULT_32_PTStackBlockage : Subsystem
  Manual Switch1 : ManualSwitch
  Manual Switch2 : ManualSwitch
  Manual Switch7 : ManualSwitch
  Mux1 : Mux  Inputs=2
  Mux2 : Mux  Inputs=2
  N=4901 rpm1 : Constant  Value=4901
  Product1 : Product  RndMeth=Zero
  Product2 : Product  Inputs=*/  RndMeth=Zero
  Scope{1..4} (4 alike) : Scope  Commented=on
  Sum : Sum  Inputs=|-+
  Sum1 : Sum  Inputs=+-|
  Sum{2..3,9..10} (4 alike) : Sum  Inputs=|+-
  Sum4 : Sum  Inputs=|++
  To Workspace : ToWorkspace  VariableName=zz_data_PTEff  SampleTime=0.2
  efficiency : Fcn  Expr=(u-340)/(340)*(0.126)+0.863
  hot_air : Subsystem
  i : Integrator  InitialCondition=340  LimitOutput=on  UpperSaturationLimit=1000  LowerSaturationLimit=1
  i1 : Integrator  InitialCondition=203  LimitOutput=on  UpperSaturationLimit=500  LowerSaturationLimit=1
  i2 : Integrator  InitialCondition=1082  LimitOutput=on  UpperSaturationLimit=2000  LowerSaturationLimit=400
  k= Cp(P,T) /(Cp(P,T)-R) : Fcn  Expr=u(1)/(u(1)-0.287)
  offset compensator : Fcn  Expr=(u-85)/(85)*(11.25)+11.25  SampleTime=1
  power : Math  Operator=pow  SignedPower=on
  pressure loss 13.0 kPa : Constant  Value=13
  s1 : Constant  Value=203.383
  s2 : Constant  Value=0.847928
  tc = 1 : Gain
  tc = 16 : Gain  Gain=1/16
  temp time constant : Gain  Gain=1/2
  trb_ex_press : Outport
  trb_ex_temp : Outport  Port=2
  wires:
  ../1 -> power/1
  turbine_inlet_press/1 -> Sum3/1
  tc = 16/1 -> i1/1
  Sum2/1 -> tc = 16/1
  i1/1 -> 0.5973/1, Sum2/2
  s2/1 -> Mux1/1
  Mux1/1 -> Scope4/1
  i2/1 -> Sum10/2, Sum4/1, Scope1/1
  10 ~ 2000/1 -> Sum10/1
  temp gas/1 -> hot_air/1(Tinlet), Product1/2
  Sum1/1 -> Product1/1
  Constant2/1 -> Sum1/1
  Product1/1 -> 10 ~ 2000/1
  temp time constant/1 -> i2/1
  Sum10/1 -> temp time constant/1
  tc = 1/1 -> i/1
  Sum9/1 -> tc = 1/1
  Sum/1 -> -/2
  (k-1)/k/1 -> power/2
  hot_air/1(Cp(P1,T1)) -> k= Cp(P,T) /(Cp(P,T)-R)/1
  k= Cp(P,T) /(Cp(P,T)-R)/1 -> (k-1)/k/1
  Sum3/1 -> Sum9/1, Scope3/1, Delay = 3.4/1
  -/1 -> Sum1/2
  Constant1/1 -> Sum/2
  power/1 -> Sum/1
  i/1 -> efficiency/1, ../1, Sum9/2
  s1/1 -> Mux2/1
  Mux2/1 -> Scope2/1
  offset compensator/1 -> Sum4/2
  hot_gas_flow/1 -> offset compensator/1
  Sum4/1 -> trb_ex_temp/1
  0.5973/1 -> trb_ex_press/1, Mux2/2, ../2
  N=4901 rpm1/1 -> Product2/2
  [pwrtrb_fr_rpm] -> Product2/1
  Product2/1 -> -1/1
  -1/1 -> Mux1/2, -/1
  Delay = 3.4/1 -> Sum2/1
  FAULT_26_PTFouling/1(Out1) -> Manual Switch7/1
  FAULT_27_PTBladeDamage/1(Out1) -> Manual Switch1/1
  Manual Switch7/1 -> Manual Switch1/2, FAULT_27_PTBladeDamage/1(In1)
  efficiency/1 -> FAULT_26_PTFouling/1(In1), Manual Switch7/2
  Manual Switch1/1 -> -1/2, To Workspace/1
  FAULT_32_PTStackBlockage/1(Out1) -> Manual Switch2/1
  pressure loss 13.0 kPa/1 -> Manual Switch2/2, FAULT_32_PTStackBlockage/1(In1)
  Manual Switch2/1 -> Sum3/2

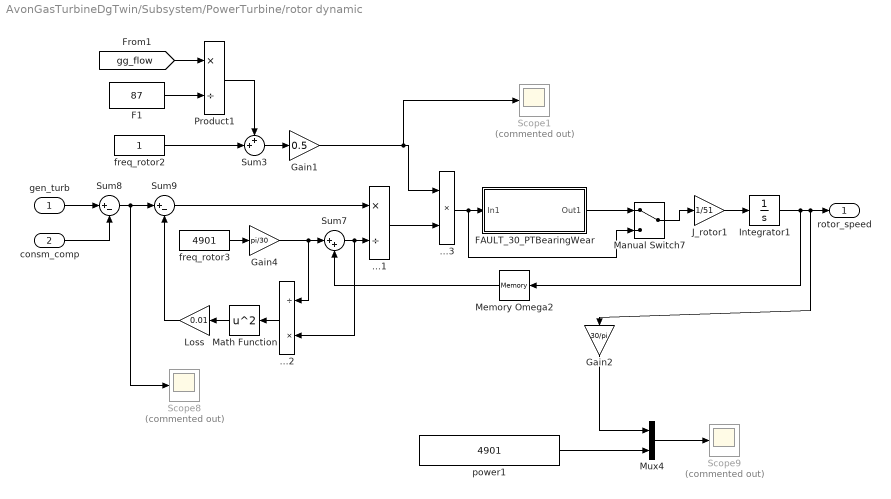
== system AvonGasTurbineDgTwin/Subsystem/PowerTurbine/rotor dynamic ==
  gen_turb : Inport
  consm_comp : Inport  Port=2
  ...1 : Product  Inputs=*/
  ...2 : Product  Inputs=/*
  ...3 : Product
  F1 : Constant  Value=87
  FAULT_30_PTBearingWear : Subsystem
  Gain1 : Gain  Gain=0.5
  Gain2 : Gain  Gain=30/pi
  Gain4 : Gain  Gain=pi/30
  Integrator1 : Integrator  InitialCondition=pi/30*4901  LimitOutput=on  UpperSaturationLimit=4900*1.20  LowerSaturationLimit=0.01
  J_rotor1 : Gain  Gain=1/51
  Loss : Gain  Gain=0.01
  Manual Switch7 : ManualSwitch
  Math Function : Math  Operator=square  SignedPower=on
  Memory Omega2 : Memory  InitialCondition=pi/30*4901
  Mux4 : Mux  Inputs=2
  Product1 : Product  Inputs=*/
  Scope1 : Scope  Commented=on
  Scope8 : Scope  Commented=on
  Scope9 : Scope  Commented=on
  Sum3 : Sum  Inputs=++|
  Sum7 : Sum  Inputs=|++
  Sum8 : Sum  Inputs=|+-
  Sum9 : Sum  Inputs=|+-
  freq_rotor2 : Constant
  freq_rotor3 : Constant  Value=4901
  power1 : Constant  Value=4901
  rotor_speed : Outport
  wires:
  Sum9/1 -> ...1/1
  Memory Omega2/1 -> Sum7/2
  Gain4/1 -> ...2/1, Sum7/1
  Sum7/1 -> ...2/2, ...1/2
  ...1/1 -> ...3/2
  J_rotor1/1 -> Integrator1/1
  Loss/1 -> Sum9/2
  consm_comp/1 -> Sum8/2
  Sum8/1 -> Scope8/1, Sum9/1
  ...2/1 -> Math Function/1
  Gain1/1 -> ...3/1, Scope1/1
  Math Function/1 -> Loss/1
  Integrator1/1 -> Memory Omega2/1, rotor_speed/1, Gain2/1
  power1/1 -> Mux4/2
  Mux4/1 -> Scope9/1
  Gain2/1 -> Mux4/1
  gen_turb/1 -> Sum8/1
  freq_rotor3/1 -> Gain4/1
  F1/1 -> Product1/2
  [gg_flow] -> Product1/1
  Product1/1 -> Sum3/1
  freq_rotor2/1 -> Sum3/2
  Sum3/1 -> Gain1/1
  FAULT_30_PTBearingWear/1(Out1) -> Manual Switch7/1
  ...3/1 -> Manual Switch7/2, FAULT_30_PTBearingWear/1(In1)
  Manual Switch7/1 -> J_rotor1/1

== system AvonGasTurbineDgTwin/Subsystem/comp_temp1/Air_Intake ==
  In1 : Inport
  Filter Constant : Constant  Value=0.0003
  Product : Product
  Scope : Scope  Commented=on
  Square : Math  Operator=square
  deltaP : Outport
  wires:
  In1/1 -> Square/1
  Filter Constant/1 -> Product/1
  Square/1 -> Scope/1, Product/2
  Product/1 -> deltaP/1

== system AvonGasTurbineDgTwin/Subsystem/comp_temp1/Cp @Cop Outlet ==
  Tinlet : Inport
  Cp : Fcn  Expr=(3.355+5.75*1e-4*u(1)-1600*u(1)^(-2))*0.28714  SampleTime=1
  oC-----> K : Fcn  Expr=(u(1)+273.15)  SampleTime=1
  Cp(T) : Outport
  wires:
  oC-----> K/1 -> Cp/1
  Cp/1 -> Cp(T)/1
  Tinlet/1 -> oC-----> K/1

== system AvonGasTurbineDgTwin/Subsystem/comp_temp1/Cp_com_in ==
  humidity ratio : Inport
  pressuer : Inport  Port=2
  temp. : Inport  Port=3
  .1 : Product  RndMeth=Zero
  .2 : Product  RndMeth=Zero
  Cp dry air : Subsystem
  Cp steam : Subsystem
  R dry air : Constant  Value=0.287
  R steam : Constant  Value=0.4615
  Specific humidity : Subsystem
  Sum1 : Sum  Inputs=++|
  Sum4 : Sum  Inputs=|++
  Cp : Outport
  Rwet : Outport  Port=2
  wires:
  .1/1 -> Sum4/1
  Specific humidity/1(y) -> .2/2, .1/1
  Cp steam/1(Cp(T)) -> .1/2
  Cp dry air/1(Cp(T)) -> Sum4/2
  humidity ratio/1 -> Specific humidity/1(humidity)
  pressuer/1 -> Specific humidity/2(Press_kPa)
  Sum4/1 -> Cp/1
  temp./1 -> Specific humidity/3(temp), Cp steam/1(Tinlet), Cp dry air/1(Tinlet)
  R steam/1 -> .2/1
  .2/1 -> Sum1/2
  Sum1/1 -> Rwet/1
  R dry air/1 -> Sum1/1

== system AvonGasTurbineDgTwin/Subsystem/comp_temp1/FAULT_01_AirIntakeFilterFouling ==
  deltaP : Inport
  FAULT_01_multiplier : FromWorkspace  VariableName=FAULT_01_multiplier  SampleTime=-1
  Mux : Mux  Inputs=2
  Product : Product
  Scope{,1..3} (4 alike) : Scope  Commented=on
  Out1 : Outport
  wires:
  FAULT_01_multiplier/1 -> Product/1, Scope/1
  deltaP/1 -> Scope1/1, Mux/2, Product/2
  Product/1 -> Mux/1, Scope2/1, Out1/1
  Mux/1 -> Scope3/1

== system AvonGasTurbineDgTwin/Subsystem/comp_temp1/FAULT_02_CompBladeFouling ==
  In1 : Inport
  FAULT_02_multiplier : FromWorkspace  VariableName=FAULT_02_multiplier  SampleTime=-1
  Mux : Mux  Inputs=2
  Product : Product
  Scope{,1..3} (4 alike) : Scope  Commented=on
  Out1 : Outport
  wires:
  FAULT_02_multiplier/1 -> Product/1, Scope/1
  In1/1 -> Scope1/1, Mux/2, Product/2
  Product/1 -> Mux/1, Scope2/1, Out1/1
  Mux/1 -> Scope3/1

== system AvonGasTurbineDgTwin/Subsystem/comp_temp1/FAULT_03_CompBladeDamage ==
  In1 : Inport
  FAULT_03_multiplier : FromWorkspace  VariableName=FAULT_03_multiplier  SampleTime=-1
  Mux : Mux  Inputs=2
  Product : Product
  Scope{,1..3} (4 alike) : Scope  Commented=on
  Out1 : Outport
  wires:
  FAULT_03_multiplier/1 -> Product/1, Scope/1
  In1/1 -> Scope1/1, Mux/2, Product/2
  Product/1 -> Mux/1, Scope2/1, Out1/1
  Mux/1 -> Scope3/1

== system AvonGasTurbineDgTwin/Subsystem/comp_temp1/FAULT_04_CompSurgeStall ==
  In1 : Inport
  FAULT_04_multiplier : FromWorkspace  VariableName=FAULT_04_multiplier  SampleTime=-1
  Mux : Mux  Inputs=2
  Product : Product
  Scope{,1..3} (4 alike) : Scope  Commented=on
  Out1 : Outport
  wires:
  FAULT_04_multiplier/1 -> Product/1, Scope/1
  In1/1 -> Scope1/1, Mux/2, Product/2
  Product/1 -> Mux/1, Scope2/1, Out1/1
  Mux/1 -> Scope3/1

== system AvonGasTurbineDgTwin/Subsystem/comp_temp1/FAULT_05_DiffuserDamage ==
  In1 : Inport
  FAULT_05_multiplier : FromWorkspace  VariableName=FAULT_05_multiplier  SampleTime=-1
  Mux : Mux  Inputs=2
  Product : Product
  Scope{,1..3} (4 alike) : Scope  Commented=on
  Out1 : Outport
  wires:
  FAULT_05_multiplier/1 -> Product/1, Scope/1
  In1/1 -> Scope1/1, Mux/2, Product/2
  Product/1 -> Mux/1, Scope2/1, Out1/1
  Mux/1 -> Scope3/1

== system AvonGasTurbineDgTwin/Subsystem/Combustor1/combustion chamber 1/ Cp dry air  ==
  Tinlet : Inport
  Cp : Fcn  Expr=(3.355+5.75*1e-4*u(1)-1600*u(1)^(-2))*0.28714  SampleTime=1
  Cp(T) : Outport
  wires:
  Tinlet/1 -> Cp/1
  Cp/1 -> Cp(T)/1

== system AvonGasTurbineDgTwin/Subsystem/Combustor1/combustion chamber 1/Cp Hot Gas  ==
  Tinlet : Inport
  Cp : Fcn  Expr=(3.355+5.75*1e-4*u(1)-1600*u(1)^(-2))*0.28714  SampleTime=1
  Cp(T) : Outport
  wires:
  Tinlet/1 -> Cp/1  "Kelvin"
  Cp/1 -> Cp(T)/1

== system AvonGasTurbineDgTwin/Subsystem/Combustor1/combustion chamber 1/Cp fuel ==
  Tinlet : Inport
  Cp : Fcn  Expr=(1.702+9.081*1e-3*u(1)-2.164*1e-6*u(1)^2)*0.5183  SampleTime=1
  oC-----> K : Fcn  Expr=(u(1)+273.15)  SampleTime=1
  Cp(T) : Outport
  wires:
  oC-----> K/1 -> Cp/1
  Cp/1 -> Cp(T)/1
  Tinlet/1 -> oC-----> K/1

== system AvonGasTurbineDgTwin/Subsystem/FG MCV model1/CV model chamber 2/Cp FG ==
  Tinlet : Inport
  Cp : Fcn  Expr=(1.702+9.081*1e-3*u(1)-2.164*1e-6*u(1)^2)*0.5183  SampleTime=1
  oC-----> K : Fcn  Expr=(u(1)+273.15)  SampleTime=1
  Cp(T) : Outport
  wires:
  oC-----> K/1 -> Cp/1
  Cp/1 -> Cp(T)/1
  Tinlet/1 -> oC-----> K/1

== system AvonGasTurbineDgTwin/Subsystem/FG MCV model1/CV model chamber 2/density FG ==
  FG_prss : Inport
  FG_temp : Inport  Port=2
  1+0.257*Pr-0.533*Pr/Tr : Fcn  Expr=1+0.257*u(1)-0.533*u(1)/u(2)
  Constant3 : Constant  Value=273.15
  Mux : Mux  Inputs=2
  Sum2 : Sum  Inputs=|++
  Tcr : Constant  Value=191
  Tnormal : Constant  Value=273.15+15
  Tnormal/T : Product  Inputs=*/  RndMeth=Zero
  Zn : Constant  Value=0.9974
  density @ n.c.1 : Gain  Gain=0.78862
  density @ n.c.2 : Gain  Gain=1/14.89
  p/pcr : Product  Inputs=*/  RndMeth=Zero
  p/pnormal1 : Product  Inputs=/*  RndMeth=Zero
  p1 : Product  Inputs=3  RndMeth=Zero
  pcr : Constant  Value=4640
  pnormal2 : Constant  Value=101.3
  t/Tc : Product  Inputs=*/  RndMeth=Zero
  z correction : Product  Inputs=/*  RndMeth=Zero
  density : Outport
  wires:
  Tnormal/1 -> Tnormal/T/1
  Constant3/1 -> Sum2/2
  Sum2/1 -> Tnormal/T/2, t/Tc/1
  pcr/1 -> p/pcr/2
  Tcr/1 -> t/Tc/2
  Zn/1 -> z correction/2
  FG_temp/1 -> Sum2/1
  p/pcr/1 -> Mux/1  "pr"
  t/Tc/1 -> Mux/2  "Tr"
  density @ n.c.2/1 -> density/1
  z correction/1 -> p1/3
  Mux/1 -> 1+0.257*Pr-0.533*Pr/Tr/1
  1+0.257*Pr-0.533*Pr/Tr/1 -> z correction/1
  FG_prss/1 -> p/pnormal1/2, p/pcr/1
  pnormal2/1 -> p/pnormal1/1
  p/pnormal1/1 -> p1/2
  p1/1 -> density @ n.c.1/1
  density @ n.c.1/1 -> density @ n.c.2/1
  Tnormal/T/1 -> p1/1

== system AvonGasTurbineDgTwin/Subsystem/FG MCV model1/Subsystem1/Z ==
  T : Inport
  P : Inport  Port=2
  1+0.257*Pr-0.533*Pr/Tr1 : Fcn  Expr=1+0.257*u(1)-0.533*u(1)/u(2)
  Mux5 : Mux  Inputs=2
  Tcr1 : Constant  Value=191
  p/pcr1 : Product  Inputs=*/  RndMeth=Zero
  pcr1 : Constant  Value=4640
  t/Tc1 : Product  Inputs=*/  RndMeth=Zero
  Z : Outport
  wires:
  Mux5/1 -> 1+0.257*Pr-0.533*Pr/Tr1/1
  P/1 -> p/pcr1/1
  T/1 -> t/Tc1/1
  Tcr1/1 -> t/Tc1/2
  1+0.257*Pr-0.533*Pr/Tr1/1 -> Z/1
  t/Tc1/1 -> Mux5/2  "Tr"
  pcr1/1 -> p/pcr1/2
  p/pcr1/1 -> Mux5/1  "pr"

== system AvonGasTurbineDgTwin/Subsystem/GasGenerator/Turbine section/FAULT_21_GGTurbFouling ==
  In1 : Inport
  FAULT_21_multiplier : FromWorkspace  VariableName=FAULT_21_multiplier  SampleTime=-1
  Mux : Mux  Inputs=2
  Product : Product
  Scope{,1..3} (4 alike) : Scope  Commented=on
  Out1 : Outport
  wires:
  FAULT_21_multiplier/1 -> Product/1, Scope/1
  In1/1 -> Scope1/1, Mux/2, Product/2
  Product/1 -> Mux/1, Scope2/1, Out1/1
  Mux/1 -> Scope3/1

== system AvonGasTurbineDgTwin/Subsystem/GasGenerator/Turbine section/FAULT_22_GGTurbBladeDamage ==
  In1 : Inport
  FAULT_22_multiplier : FromWorkspace  VariableName=FAULT_22_multiplier  SampleTime=-1
  Mux : Mux  Inputs=2
  Product : Product
  Scope{,1..3} (4 alike) : Scope  Commented=on
  Out1 : Outport
  wires:
  FAULT_22_multiplier/1 -> Product/1, Scope/1
  In1/1 -> Scope1/1, Mux/2, Product/2
  Product/1 -> Mux/1, Scope2/1, Out1/1
  Mux/1 -> Scope3/1

== system AvonGasTurbineDgTwin/Subsystem/GasGenerator/Turbine section/hot_air ==
  Tinlet : Inport
  Cp(T) : Fcn  Expr=(3.355+5.75*1e-4*u(1)-1600*u(1)^(-2))*0.28714  SampleTime=1
  Cp(P1,T1) : Outport
  wires:
  Cp(T)/1 -> Cp(P1,T1)/1
  Tinlet/1 -> Cp(T)/1

== system AvonGasTurbineDgTwin/Subsystem/GasGenerator/cooling 1/Cp Temp ==
  Tinlet : Inport
  Cp : Fcn  Expr=(3.355+5.75*1e-4*u(1)-1600*u(1)^(-2))*0.28714  SampleTime=1
  Cp(T) : Outport
  wires:
  Cp/1 -> Cp(T)/1
  Tinlet/1 -> Cp/1  "Kelvin"

== system AvonGasTurbineDgTwin/Subsystem/GasGenerator/cooling 1/Cp Temp air ==
  Tinlet : Inport
  Cp : Fcn  Expr=(3.355+5.75*1e-4*u(1)-1600*u(1)^(-2))*0.28714  SampleTime=1
  Cp(T) : Outport
  wires:
  Tinlet/1 -> Cp/1  "Kelvin"
  Cp/1 -> Cp(T)/1

== system AvonGasTurbineDgTwin/Subsystem/GasGenerator/cooling 1/Cp Temp hot gas ==
  Tinlet : Inport
  Cp : Fcn  Expr=(3.355+5.75*1e-4*u(1)-1600*u(1)^(-2))*0.28714  SampleTime=1
  Cp(T) : Outport
  wires:
  Cp/1 -> Cp(T)/1
  Tinlet/1 -> Cp/1  "Kelvin"

== system AvonGasTurbineDgTwin/Subsystem/GasGenerator/cooling 2/Cp Temp ==
  Tinlet : Inport
  Cp : Fcn  Expr=(3.355+5.75*1e-4*u(1)-1600*u(1)^(-2))*0.28714  SampleTime=1
  Cp(T) : Outport
  wires:
  Tinlet/1 -> Cp/1  "Kelvin"
  Cp/1 -> Cp(T)/1

== system AvonGasTurbineDgTwin/Subsystem/GasGenerator/cooling 2/Cp Temp air ==
  Tinlet : Inport
  Cp : Fcn  Expr=(3.355+5.75*1e-4*u(1)-1600*u(1)^(-2))*0.28714  SampleTime=1
  Cp(T) : Outport
  wires:
  Cp/1 -> Cp(T)/1
  Tinlet/1 -> Cp/1  "Kelvin"

== system AvonGasTurbineDgTwin/Subsystem/GasGenerator/cooling 2/Cp Temp hot gas ==
  Tinlet : Inport
  Cp : Fcn  Expr=(3.355+5.75*1e-4*u(1)-1600*u(1)^(-2))*0.28714  SampleTime=1
  Cp(T) : Outport
  wires:
  Tinlet/1 -> Cp/1  "Kelvin"
  Cp/1 -> Cp(T)/1

== system AvonGasTurbineDgTwin/Subsystem/PowerTurbine/Turbine section/FAULT_26_PTFouling ==
  In1 : Inport
  FAULT_26_multiplier : FromWorkspace  VariableName=FAULT_26_multiplier  SampleTime=-1
  Mux : Mux  Inputs=2
  Product : Product
  Scope{,1..3} (4 alike) : Scope  Commented=on
  Out1 : Outport
  wires:
  FAULT_26_multiplier/1 -> Product/1, Scope/1
  In1/1 -> Scope1/1, Mux/2, Product/2
  Product/1 -> Mux/1, Scope2/1, Out1/1
  Mux/1 -> Scope3/1

== system AvonGasTurbineDgTwin/Subsystem/PowerTurbine/Turbine section/FAULT_27_PTBladeDamage ==
  In1 : Inport
  FAULT_27_multiplier : FromWorkspace  VariableName=FAULT_27_multiplier  SampleTime=-1
  Mux : Mux  Inputs=2
  Product : Product
  Scope{,1..3} (4 alike) : Scope  Commented=on
  Out1 : Outport
  wires:
  FAULT_27_multiplier/1 -> Product/1, Scope/1
  In1/1 -> Scope1/1, Mux/2, Product/2
  Product/1 -> Mux/1, Scope2/1, Out1/1
  Mux/1 -> Scope3/1

== system AvonGasTurbineDgTwin/Subsystem/PowerTurbine/Turbine section/FAULT_32_PTStackBlockage ==
  In1 : Inport
  FAULT_32_multiplier : FromWorkspace  VariableName=FAULT_32_multiplier  SampleTime=-1
  Mux : Mux  Inputs=2
  Product : Product
  Scope{,1..3} (4 alike) : Scope  Commented=on
  Out1 : Outport
  wires:
  FAULT_32_multiplier/1 -> Product/1, Scope/1
  In1/1 -> Scope1/1, Mux/2, Product/2
  Product/1 -> Mux/1, Scope2/1, Out1/1
  Mux/1 -> Scope3/1

== system AvonGasTurbineDgTwin/Subsystem/PowerTurbine/Turbine section/hot_air ==
  Tinlet : Inport
  Cp(T) : Fcn  Expr=(3.355+5.75*1e-4*u(1)-1600*u(1)^(-2))*0.28714  SampleTime=1
  Cp(P1,T1) : Outport
  wires:
  Tinlet/1 -> Cp(T)/1
  Cp(T)/1 -> Cp(P1,T1)/1

== system AvonGasTurbineDgTwin/Subsystem/PowerTurbine/rotor dynamic/FAULT_30_PTBearingWear ==
  In1 : Inport
  FAULT_30_multiplier : FromWorkspace  VariableName=FAULT_30_multiplier  SampleTime=-1
  Mux : Mux  Inputs=2
  Product : Product
  Scope{,1..3} (4 alike) : Scope  Commented=on
  Out1 : Outport
  wires:
  FAULT_30_multiplier/1 -> Product/1, Scope/1
  In1/1 -> Scope1/1, Mux/2, Product/2
  Product/1 -> Mux/1, Scope2/1, Out1/1
  Mux/1 -> Scope3/1

== system AvonGasTurbineDgTwin/Subsystem/comp_temp1/Cp_com_in/Cp dry air ==
  Tinlet : Inport
  Cp : Fcn  Expr=(3.355+5.75*1e-4*u(1)-1600*u(1)^(-2))*0.28714  SampleTime=1
  Cp(T) : Outport
  wires:
  Cp/1 -> Cp(T)/1
  Tinlet/1 -> Cp/1

== system AvonGasTurbineDgTwin/Subsystem/comp_temp1/Cp_com_in/Cp steam ==
  Tinlet : Inport
  Cp : Fcn  Expr=(3.47+1.45*1e-3*u(1)+1.21*1e4*u(1)^(-2))*0.4615  SampleTime=1
  Cp(T) : Outport
  wires:
  Tinlet/1 -> Cp/1
  Cp/1 -> Cp(T)/1

== system AvonGasTurbineDgTwin/Subsystem/comp_temp1/Cp_com_in/Specific humidity ==
  humidity : Inport
  Press_kPa : Inport  Port=2
  temp : Inport  Port=3
  1/100 : Gain  Gain=0.01
  Ps (saturation pressure) : Fcn  Expr=((u-200.5754)/81.4934)^6.1556  SampleTime=1
  Scope11 : Scope
  "Specific humidity " : Gain  Gain=0.6219
  Sum : Sum  Inputs=-+
  x : Product  RndMeth=Zero
  x1 : Product  Inputs=*/  RndMeth=Zero
  y : Outport
  wires:
  Ps (saturation pressure)/1 -> Scope11/1, x/1
  "Specific humidity "/1 -> y/1
  x1/1 -> "Specific humidity "/1
  Sum/1 -> x1/2
  Press_kPa/1 -> Sum/2
  x/1 -> x1/1, Sum/1  "pv"
  1/100/1 -> x/2
  humidity/1 -> 1/100/1
  temp/1 -> Ps (saturation pressure)/1
